simulink model "rfsoc4x2_ospfb_128"  (R2021a)
settings: Solver=VariableStepAuto  StartTime=0.0  StopTime=2048  RelTol=1e-3
undefined symbols (not defined in the file): pfb_coeff_gen_calc
libraries: xbsIndex_r4 x37092, casper_library_delays x737, casper_library_misc x68, xps_library x1
(part 143 of 339)

== system rfsoc4x2_ospfb_128/fft2/fft_direct/butterfly1_0 ==
  a : Inport
  b : Inport  Port=2
  sync_in : Inport  Port=3
  shift : Inport  Port=4
  Concat : xbsIndex_r4/Concat  num_inputs=2  dbl_ovrd=off  block_type=concat
  bus_add : Subsystem  AncestorBlock=casper_library_bus/bus_addsub  mask(bus_addsub){opmode=0, n_bits_a=[18 18], bin_pt_a=17, type_a=1, n_bits_b=[19 19], bin_pt_b=17, type_b=1, cmplx=on, misc=off, async=off, floating_point=off, float_type=single, exp_width=8, frac_width=24, n_bits_out=20, bin_pt_out=17, type_out=1, quantization=0, overflow=0, add_implementation=behavioral HDL, csp_latency=2, pipeline_en=off, pipeline_latency=0}
      mask prompts: opmode "mode (Addition=0, Subtraction=1)"; n_bits_a "a input bit widths"; bin_pt_a "a input binary points"; type_a "a input type (Unsigned=0, Signed=1)"; n_bits_b "b input bit widths"; bin_pt_b "b input binary points"; type_b "b input type (Unsigned=0, Signed=1)"; cmplx "complex"; misc "misc support"; async "asynchronous operation"; floating_point "floating point"; exp_width "exponent width"; frac_width "fraction width"; n_bits_out "output bit widths"; bin_pt_out "output binary points"; type_out "output type (Unsigned=0, Signed=1)"; quantization "quantization strategy (Truncate=0, Round  (unbiased: +/- Inf)=1)"; overflow "overflow strategy (Wrap=0, Saturate=1, Flag as error=2)"; add_implementation "adder implementation"; csp_latency "latency"; pipeline_en "pipeline enable"; pipeline_latency "pipeline latency"
      mask help: Add/subtract components of two busses
      mask init: same as rfsoc4x2_ospfb_128/fft2/fft_direct/butterfly0_0/bus_add
      mask Callback floating_point:
      | onoff = get_param(gcb, 'floating_point');
      | if strcmp(onoff,'on')
      |     enable_fixpt = 'off';
      |     set_param_state(gcb, 'float_type', 'on')
      | 
      |     f_type = get_param(gcb, 'float_type');
      |     if strcmp(f_type,'custom')
      |         set_param_state(gcb, 'exp_width', 'on')
      |         set_param_state(gcb, 'frac_width', 'on')
      |     else
      |         set_param_state(gcb, 'exp_width', 'off')
      |         set_param_state(gcb, 'frac_width', 'off')
      |     end
      | 
      | 
      | else
      |     enable_fixpt = 'on';
      |     set_param_state(gcb, 'float_type', 'off')
      |     set_param_state(gcb, 'exp_width', 'off')
      |     set_param_state(gcb, 'frac_width', 'off')
      | end
      | 
      | set_param_state(gcb, 'n_bits_a', enable_fixpt)
      | set_param_state(gcb, 'bin_pt_a', enable_fixpt)
      | set_param_state(gcb, 'type_a', enable_fixpt)
      | set_param_state(gcb, 'n_bits_b', enable_fixpt)
      | set_param_state(gcb, 'bin_pt_b', enable_fixpt)
      | set_param_state(gcb, 'type_b', enable_fixpt)
      | 
      | set_param_state(gcb, 'n_bits_out', enable_fixpt)
      | set_param_state(gcb, 'bin_pt_out', enable_fixpt)
      | set_param_state(gcb, 'type_out', enable_fixpt)
      | set_param_state(gcb, 'quantization', enable_fixpt)
      | set_param_state(gcb, 'overflow', enable_fixpt)
      mask TypeOptions float_type: single | custom
      mask Callback float_type:
      | f_type = get_param(gcb, 'float_type');
      | if strcmp(f_type,'custom')
      |     set_param_state(gcb, 'exp_width', 'on')
      |     set_param_state(gcb, 'frac_width', 'on')
      | else
      |     set_param_state(gcb, 'exp_width', 'off')
      |     set_param_state(gcb, 'frac_width', 'off')
      | end
      mask TypeOptions add_implementation: behavioral HDL | fabric core | DSP48 core
  bus_convert : Subsystem  AncestorBlock=casper_library_bus/bus_convert  mask(bus_convert){n_bits_in=[21 21 21 21], bin_pt_in=[18 18 18 18], cmplx=on, n_bits_out=18, bin_pt_out=17, quantization=1, overflow=0, csp_latency=conv_latency, of=on, misc=off}
      mask prompts: n_bits_in "input bit widths"; bin_pt_in "input binary points"; cmplx "input complex"; n_bits_out "output bit widths"; bin_pt_out "output binary points"; quantization "quantization strategy (Truncate=0, Round  (unbiased: +/- Inf)=1, Round (unbiased: Even Values)=2)"; overflow "overflow strategy (Wrap=0, Saturate=1, Flag as error=2)"; csp_latency "latency"; of "overflow indication"; misc "misc support"
      mask help: Convert components of busses
      mask init: same as rfsoc4x2_ospfb_128/fft2/fft_direct/butterfly0_0/bus_convert
  bus_expand : Subsystem  AncestorBlock=casper_library_flow_control/bus_expand  mask(bus_expand){mode=divisions of equal size, outputNum=2, outputWidth=[72 72], outputBinaryPt=[0,0], outputArithmeticType=[0,0], show_format=off, outputToWorkspace=off, variablePrefix=out, outputToModelAsWell=on}
      mask prompts: outputNum "Number of outputs:"; outputWidth "Output width:"; outputBinaryPt "Output binary point position:"; outputArithmeticType "Output arithmetic type (ufix=0, fix=1, bool=2):"; show_format "Print format string?"; outputToWorkspace "Output to workspace?"; variablePrefix "Variable name prefix:"; outputToModelAsWell "Output to model as well?"
      mask help:
      | Expands a 'bus' made using a bus_create or Xilinx
      | concat block.
      | The input will be divided into the specified number
      | of outputs with the specified arithmetic types.
      | Divisions are made from most significant bit.
      mask init: same as rfsoc4x2_ospfb_128/bus_expand1
      settings: AttributesFormatString=2 outputs
      mask TypeOptions mode: divisions of equal size | divisions of arbitrary size
      mask Callback mode: %bus_expand_callback();
      mask Callback outputWidth: %bus_expand_callback();
      mask Callback outputToWorkspace: %bus_expand_callback();
  bus_norm0 : Subsystem  AncestorBlock=casper_library_bus/bus_convert  mask(bus_convert){n_bits_in=[20 20 20 20], bin_pt_in=[17 17 17 17], cmplx=on, n_bits_out=21, bin_pt_out=18, quantization=0, overflow=0, csp_latency=0, of=off, misc=off}
      mask prompts: n_bits_in "input bit widths"; bin_pt_in "input binary points"; cmplx "input complex"; n_bits_out "output bit widths"; bin_pt_out "output binary points"; quantization "quantization strategy (Truncate=0, Round  (unbiased: +/- Inf)=1, Round (unbiased: Even Values)=2)"; overflow "overflow strategy (Wrap=0, Saturate=1, Flag as error=2)"; csp_latency "latency"; of "overflow indication"; misc "misc support"
      mask help: Convert components of busses
      mask init: same as rfsoc4x2_ospfb_128/fft2/fft_direct/butterfly0_0/bus_convert
  bus_norm1 : Subsystem  AncestorBlock=casper_library_bus/bus_convert  mask(bus_convert){n_bits_in=[20 20 20 20], bin_pt_in=[18 18 18 18], cmplx=on, n_bits_out=21, bin_pt_out=18, quantization=0, overflow=0, csp_latency=0, of=off, misc=off}
      mask prompts: n_bits_in "input bit widths"; bin_pt_in "input binary points"; cmplx "input complex"; n_bits_out "output bit widths"; bin_pt_out "output binary points"; quantization "quantization strategy (Truncate=0, Round  (unbiased: +/- Inf)=1, Round (unbiased: Even Values)=2)"; overflow "overflow strategy (Wrap=0, Saturate=1, Flag as error=2)"; csp_latency "latency"; of "overflow indication"; misc "misc support"
      mask help: Convert components of busses
      mask init: same as rfsoc4x2_ospfb_128/fft2/fft_direct/butterfly0_0/bus_convert
  bus_relational : Subsystem  AncestorBlock=casper_library_bus/bus_relational  mask(bus_relational){n_bits_a=4, bin_pt_a=0, type_a=0, n_bits_b=[4 4], bin_pt_b=0, type_b=0, en=off, misc=off, mode=a!=b, csp_latency=1}
      mask prompts: n_bits_a "a input bit widths"; bin_pt_a "a input binary points"; type_a "a input type (Unsigned=0, Signed=1)"; n_bits_b "b input bit widths"; bin_pt_b "b input binary points"; type_b "b input type (Unsigned=0, Signed=1)"; en "en port"; misc "misc support"; mode "comparison:"; csp_latency "latency"
      mask help: Find the relational product of two busses
      mask init: same as rfsoc4x2_ospfb_128/fft2/fft_direct/butterfly0_0/bus_relational
      mask TypeOptions mode: a=b | a!=b | a<b | a>b | a<=b | a>=b
  bus_scale : Subsystem  AncestorBlock=casper_library_bus/bus_scale  mask(bus_scale){n_bits_in=[20 20 20 20], bin_pt_in=17, type_in=1, cmplx=on, scale_factor=-1, misc=off}
      mask prompts: n_bits_in "input bit widths"; bin_pt_in "input binary points"; type_in "input types"; cmplx "input complex"; scale_factor "scale factor (2^?)"; misc "misc support"
      mask help: Convert components of busses
      mask init:
      | bus_scale_init(gcb, ...
      |     'n_bits_in', n_bits_in, ...
      |     'bin_pt_in', bin_pt_in, ...
      |     'type_in', type_in, ...
      |     'cmplx', cmplx, ...
      |     'scale_factor', scale_factor, ...
      |     'misc', misc);
  bus_sub : Subsystem  AncestorBlock=casper_library_bus/bus_addsub  mask(bus_addsub){opmode=1, n_bits_a=[18 18], bin_pt_a=17, type_a=1, n_bits_b=[19 19], bin_pt_b=17, type_b=1, cmplx=on, misc=off, async=off, floating_point=off, float_type=single, exp_width=8, frac_width=24, n_bits_out=20, bin_pt_out=17, type_out=1, quantization=0, overflow=0, add_implementation=behavioral HDL, csp_latency=2, pipeline_en=off, pipeline_latency=0}
      mask prompts: opmode "mode (Addition=0, Subtraction=1)"; n_bits_a "a input bit widths"; bin_pt_a "a input binary points"; type_a "a input type (Unsigned=0, Signed=1)"; n_bits_b "b input bit widths"; bin_pt_b "b input binary points"; type_b "b input type (Unsigned=0, Signed=1)"; cmplx "complex"; misc "misc support"; async "asynchronous operation"; floating_point "floating point"; exp_width "exponent width"; frac_width "fraction width"; n_bits_out "output bit widths"; bin_pt_out "output binary points"; type_out "output type (Unsigned=0, Signed=1)"; quantization "quantization strategy (Truncate=0, Round  (unbiased: +/- Inf)=1)"; overflow "overflow strategy (Wrap=0, Saturate=1, Flag as error=2)"; add_implementation "adder implementation"; csp_latency "latency"; pipeline_en "pipeline enable"; pipeline_latency "pipeline latency"
      mask help: Add/subtract components of two busses
      mask init: same as rfsoc4x2_ospfb_128/fft2/fft_direct/butterfly0_0/bus_add
      mask Callback floating_point:
      | onoff = get_param(gcb, 'floating_point');
      | if strcmp(onoff,'on')
      |     enable_fixpt = 'off';
      |     set_param_state(gcb, 'float_type', 'on')
      | 
      |     f_type = get_param(gcb, 'float_type');
      |     if strcmp(f_type,'custom')
      |         set_param_state(gcb, 'exp_width', 'on')
      |         set_param_state(gcb, 'frac_width', 'on')
      |     else
      |         set_param_state(gcb, 'exp_width', 'off')
      |         set_param_state(gcb, 'frac_width', 'off')
      |     end
      | 
      | 
      | else
      |     enable_fixpt = 'on';
      |     set_param_state(gcb, 'float_type', 'off')
      |     set_param_state(gcb, 'exp_width', 'off')
      |     set_param_state(gcb, 'frac_width', 'off')
      | end
      | 
      | set_param_state(gcb, 'n_bits_a', enable_fixpt)
      | set_param_state(gcb, 'bin_pt_a', enable_fixpt)
      | set_param_state(gcb, 'type_a', enable_fixpt)
      | set_param_state(gcb, 'n_bits_b', enable_fixpt)
      | set_param_state(gcb, 'bin_pt_b', enable_fixpt)
      | set_param_state(gcb, 'type_b', enable_fixpt)
      | 
      | set_param_state(gcb, 'n_bits_out', enable_fixpt)
      | set_param_state(gcb, 'bin_pt_out', enable_fixpt)
      | set_param_state(gcb, 'type_out', enable_fixpt)
      | set_param_state(gcb, 'quantization', enable_fixpt)
      | set_param_state(gcb, 'overflow', enable_fixpt)
      mask TypeOptions float_type: single | custom
      mask Callback float_type:
      | f_type = get_param(gcb, 'float_type');
      | if strcmp(f_type,'custom')
      |     set_param_state(gcb, 'exp_width', 'on')
      |     set_param_state(gcb, 'frac_width', 'on')
      | else
      |     set_param_state(gcb, 'exp_width', 'off')
      |     set_param_state(gcb, 'frac_width', 'off')
      | end
      mask TypeOptions add_implementation: behavioral HDL | fabric core | DSP48 core
  constant : xbsIndex_r4/Constant  const=0  gui_display_data_type=Fixed-point  arith_type=Unsigned  n_bits=4  bin_pt=0  preci_type=Single  exp_width=8  frac_width=24  explicit_period=on  period=1  equ=P=C  opselect=C  inp2=PCIN>>17  opr=+  inp1=P  carry=CIN  dbl_ovrd=off  block_type=constant
  delay0 : xbsIndex_r4/Delay  rst=off  infoeditControl=Selection of Reset will increase slice count due to use of real FFs and instead of SRLs  en=off  latency=add_latency+1+conv_latency  reg_retiming=on  dbl_ovrd=off  block_type=delay
  munge : Subsystem  AncestorBlock=casper_library_flow_control/munge  mask(munge){divisions=4, div_size=[2 2 2 2], order=[0 2 1 3], arith_type_out=Unsigned, bin_pt_out=0}
      mask prompts: divisions "Number of divisions"; div_size "Division size (bits)"; order "Division packing order"; arith_type_out "Output arithmetic type"; bin_pt_out "Output binary point"
      mask help: Splits an input bus into the specified number of divisions and then recombines them in the order specified (most significant division = 0,least = number divisions-1)
      mask init:
      | munge_init(gcb, ...
      |     'divisions', divisions, ...
      |     'div_size', div_size, ...
      |     'order', order, ...
      |     'arith_type_out', arith_type_out, ...
      |     'bin_pt_out', bin_pt_out);
      settings: AttributesFormatString=|
      | split:[2 2 2 2]
      | join:[0 2 1 3]
      | Unsigned [8,0]
      mask TypeOptions arith_type_out: Unsigned | Signed  (2's comp) | Floating-point
  mux : Subsystem  AncestorBlock=casper_library_bus/bus_mux  mask(bus_mux){n_inputs=2, n_bits=[21 21 21 21 21 21 21 21], cmplx=off, misc=off, mux_latency=1}
      mask prompts: n_inputs "number of inputs"; n_bits "input bit widths"; cmplx "complex data"; misc "misc support"; mux_latency "mux latency"
      mask help: Mux components of bus
      mask init:
      | bus_mux_init(gcb, ...
      |     'n_inputs', n_inputs, ...
      |     'n_bits', n_bits, ...
      |     'cmplx', cmplx, ...
      |     'misc', misc, ...
      |     'mux_latency', mux_latency);
  shift_replicate : Subsystem  AncestorBlock=casper_library_bus/bus_replicate  mask(bus_replicate){replication=8, csp_latency=1, misc=off, implementation=core}
      mask prompts: replication "replication factor"; csp_latency "latency"; misc "misc support"; implementation "delay implementation"
      mask help: Output bus formed by replicating input bus a number of times
      mask init:
      | bus_replicate_init(gcb, ...
      |     'replication', replication, ...
      |     'csp_latency', csp_latency, ...
      |     'implementation', implementation, ...
      |     'misc', misc);
      mask TypeOptions implementation: core | behavioral
  twiddle : Subsystem  AncestorBlock=casper_library_ffts_twiddle/twiddle_general  mask(twiddle_general){n_inputs=2, FFTSize=9, Coeffs=[0 64 32 96 16 80 48 112 8 72 40 104 24 88 56 120 4 68 36 100 20 84 52 116 12 76 44 108 28 92 60 124 2 66 34 98 18 82 50 114 10 74 42 106 26 90 58 122 6 70 38 102 22 86 54 118 14 78 46 110 30 94 62 126], StepPeriod=0, coeff_bit_width=18, input_bit_width=18, bin_pt_in=17, async=off, floating_point=off, float_type=single, exp_width=8, frac_width=24, add_latency=2, mult_latency=2, bram_latency=2, conv_latency=1, add_pipe_latency=0, mult_pipe_latency=0, coeffs_bit_limit=9, coeff_sharing=off, coeff_decimation=off, coeff_generation=on, cal_bits=9, n_bits_rotation=25, max_fanout=4, use_hdl=on, use_embedded=off, quantization=Round  (unbiased: +/- Inf), overflow=Wrap}
      mask prompts: n_inputs "Number inputs"; FFTSize "FFT Size (2^?)"; Coeffs "Coefficients:"; StepPeriod "Coefficient Step Period (2^?)"; coeff_bit_width "Coefficient Bit Width"; input_bit_width "Input Bit Width"; bin_pt_in "Input binary point"; async "Asynchronous operation"; floating_point "floating point"; float_type "float type"; exp_width "exponent width"; frac_width "fraction width"; add_latency "Add Latency"; mult_latency "Mult Latency"; bram_latency "BRAM Latency"; conv_latency "Convert Latency"; add_pipe_latency "Add Pipeline Latency"; mult_pipe_latency "CMult Pipeline Latency"; coeffs_bit_limit "Number bits above which to store stage's coefficients in BRAM (2^? bits)"; coeff_sharing "BRAM sharing in coeff storage"; coeff_decimation "Store a fraction of coeff factors where useful"; coeff_generation "Generate coeffs with multipliers where useful"; cal_bits "Number calibration locations when generating coeffs (2^?)"; n_bits_rotation "Feedback rotation vector resolution"; max_fanout "Maximum fanout"; use_hdl "Use behavioural HDL for multipliers"; use_embedded "Use embedded multipliers"; quantization "Quantization Behavior"; overflow "Overflow Behavior"
      mask help: Used in biplex pipelined FFT.
      mask init: same as rfsoc4x2_ospfb_128/fft2/fft_direct/butterfly0_0/twiddle
      settings: AttributesFormatString=|
      | data=(18,17)
      | coeffs=(18,17)
      | (Round  (unbiased: +/- Inf),Wrap)
      mask Callback floating_point:
      | onoff = get_param(gcb, 'floating_point');
      | if strcmp(onoff,'on')
      |     enable_fixpt = 'off';
      |     set_param_state(gcb, 'float_type', 'on')
      | 
      |     f_type = get_param(gcb, 'float_type');
      |     if strcmp(f_type,'custom')
      |         set_param_state(gcb, 'exp_width', 'on')
      |         set_param_state(gcb, 'frac_width', 'on')
      |     else
      |         set_param_state(gcb, 'exp_width', 'off')
      |         set_param_state(gcb, 'frac_width', 'off')
      |     end
      | 
      | 
      | else
      |     enable_fixpt = 'on';
      |     set_param_state(gcb, 'float_type', 'off')
      |     set_param_state(gcb, 'exp_width', 'off')
      |     set_param_state(gcb, 'frac_width', 'off')
      | end
      | 
      | set_param_state(gcb, 'input_bit_width', enable_fixpt)
      | set_param_state(gcb, 'bin_pt_in', enable_fixpt)
      | set_param_state(gcb, 'coeff_bit_width', enable_fixpt)
      mask TypeOptions float_type: single | custom
      mask Callback float_type:
      | f_type = get_param(gcb, 'float_type');
      | if strcmp(f_type,'custom')
      |     set_param_state(gcb, 'exp_width', 'on')
      |     set_param_state(gcb, 'frac_width', 'on')
      | else
      |     set_param_state(gcb, 'exp_width', 'off')
      |     set_param_state(gcb, 'frac_width', 'off')
      | end
      mask Callback use_hdl: twiddle_general_callback(gcb);
      mask TypeOptions quantization: Truncate | Round  (unbiased: +/- Inf) | Round  (unbiased: Even Values)
      mask TypeOptions overflow: Wrap | Saturate | Error
      mask DialogControl ParameterTabVar0 Prompt: Basic
      mask DialogControl ParameterTabVar01 Prompt: Latency
      mask DialogControl ParameterTabVar012 Prompt: Implementation
  a+bw : Outport
  a-bw : Outport  Port=2
  of : Outport  Port=3
  sync_out : Outport  Port=4
  wires:
  delay0/1 -> sync_out/1
  twiddle/3(sync_out) -> delay0/1
  bus_relational/1(a!=b) -> of/1
  munge/1(dout) -> bus_relational/2(b)
  constant/1 -> bus_relational/1(a)
  bus_convert/2(overflow) -> munge/1(din)
  bus_expand/2(lsb_out1) -> a-bw/1
  bus_expand/1(msb_out2) -> a+bw/1
  bus_convert/1(dout) -> bus_expand/1(bus_in)
  mux/1(out) -> bus_convert/1(din)
  bus_norm1/1(dout) -> mux/3(d1)
  bus_norm0/1(dout) -> mux/2(d0)
  shift_replicate/1(out) -> mux/1(sel)
  bus_scale/1(dout) -> bus_norm1/1(din)
  Concat/1 -> bus_scale/1(din), bus_norm0/1(din)
  shift/1 -> shift_replicate/1(in)
  bus_sub/1(dout) -> Concat/2
  bus_add/1(dout) -> Concat/1
  twiddle/2(bwo) -> bus_sub/2(b), bus_add/2(b)
  twiddle/1(ao) -> bus_sub/1(a), bus_add/1(a)
  sync_in/1 -> twiddle/3(sync_in)
  b/1 -> twiddle/2(bi)
  a/1 -> twiddle/1(ai)

== system rfsoc4x2_ospfb_128/fft2/fft_direct/butterfly1_1 ==
  a : Inport
  b : Inport  Port=2
  sync_in : Inport  Port=3
  shift : Inport  Port=4
  Concat : xbsIndex_r4/Concat  num_inputs=2  dbl_ovrd=off  block_type=concat
  bus_add : Subsystem  AncestorBlock=casper_library_bus/bus_addsub  mask(bus_addsub){opmode=0, n_bits_a=[18 18], bin_pt_a=17, type_a=1, n_bits_b=[19 19], bin_pt_b=17, type_b=1, cmplx=on, misc=off, async=off, floating_point=off, float_type=single, exp_width=8, frac_width=24, n_bits_out=20, bin_pt_out=17, type_out=1, quantization=0, overflow=0, add_implementation=behavioral HDL, csp_latency=2, pipeline_en=off, pipeline_latency=0}
      mask prompts: opmode "mode (Addition=0, Subtraction=1)"; n_bits_a "a input bit widths"; bin_pt_a "a input binary points"; type_a "a input type (Unsigned=0, Signed=1)"; n_bits_b "b input bit widths"; bin_pt_b "b input binary points"; type_b "b input type (Unsigned=0, Signed=1)"; cmplx "complex"; misc "misc support"; async "asynchronous operation"; floating_point "floating point"; exp_width "exponent width"; frac_width "fraction width"; n_bits_out "output bit widths"; bin_pt_out "output binary points"; type_out "output type (Unsigned=0, Signed=1)"; quantization "quantization strategy (Truncate=0, Round  (unbiased: +/- Inf)=1)"; overflow "overflow strategy (Wrap=0, Saturate=1, Flag as error=2)"; add_implementation "adder implementation"; csp_latency "latency"; pipeline_en "pipeline enable"; pipeline_latency "pipeline latency"
      mask help: Add/subtract components of two busses
      mask init: same as rfsoc4x2_ospfb_128/fft2/fft_direct/butterfly0_0/bus_add
      mask Callback floating_point:
      | onoff = get_param(gcb, 'floating_point');
      | if strcmp(onoff,'on')
      |     enable_fixpt = 'off';
      |     set_param_state(gcb, 'float_type', 'on')
      | 
      |     f_type = get_param(gcb, 'float_type');
      |     if strcmp(f_type,'custom')
      |         set_param_state(gcb, 'exp_width', 'on')
      |         set_param_state(gcb, 'frac_width', 'on')
      |     else
      |         set_param_state(gcb, 'exp_width', 'off')
      |         set_param_state(gcb, 'frac_width', 'off')
      |     end
      | 
      | 
      | else
      |     enable_fixpt = 'on';
      |     set_param_state(gcb, 'float_type', 'off')
      |     set_param_state(gcb, 'exp_width', 'off')
      |     set_param_state(gcb, 'frac_width', 'off')
      | end
      | 
      | set_param_state(gcb, 'n_bits_a', enable_fixpt)
      | set_param_state(gcb, 'bin_pt_a', enable_fixpt)
      | set_param_state(gcb, 'type_a', enable_fixpt)
      | set_param_state(gcb, 'n_bits_b', enable_fixpt)
      | set_param_state(gcb, 'bin_pt_b', enable_fixpt)
      | set_param_state(gcb, 'type_b', enable_fixpt)
      | 
      | set_param_state(gcb, 'n_bits_out', enable_fixpt)
      | set_param_state(gcb, 'bin_pt_out', enable_fixpt)
      | set_param_state(gcb, 'type_out', enable_fixpt)
      | set_param_state(gcb, 'quantization', enable_fixpt)
      | set_param_state(gcb, 'overflow', enable_fixpt)
      mask TypeOptions float_type: single | custom
      mask Callback float_type:
      | f_type = get_param(gcb, 'float_type');
      | if strcmp(f_type,'custom')
      |     set_param_state(gcb, 'exp_width', 'on')
      |     set_param_state(gcb, 'frac_width', 'on')
      | else
      |     set_param_state(gcb, 'exp_width', 'off')
      |     set_param_state(gcb, 'frac_width', 'off')
      | end
      mask TypeOptions add_implementation: behavioral HDL | fabric core | DSP48 core
  bus_convert : Subsystem  AncestorBlock=casper_library_bus/bus_convert  mask(bus_convert){n_bits_in=[21 21 21 21], bin_pt_in=[18 18 18 18], cmplx=on, n_bits_out=18, bin_pt_out=17, quantization=1, overflow=0, csp_latency=conv_latency, of=on, misc=off}
      mask prompts: n_bits_in "input bit widths"; bin_pt_in "input binary points"; cmplx "input complex"; n_bits_out "output bit widths"; bin_pt_out "output binary points"; quantization "quantization strategy (Truncate=0, Round  (unbiased: +/- Inf)=1, Round (unbiased: Even Values)=2)"; overflow "overflow strategy (Wrap=0, Saturate=1, Flag as error=2)"; csp_latency "latency"; of "overflow indication"; misc "misc support"
      mask help: Convert components of busses
      mask init: same as rfsoc4x2_ospfb_128/fft2/fft_direct/butterfly0_0/bus_convert
  bus_expand : Subsystem  AncestorBlock=casper_library_flow_control/bus_expand  mask(bus_expand){mode=divisions of equal size, outputNum=2, outputWidth=[72 72], outputBinaryPt=[0,0], outputArithmeticType=[0,0], show_format=off, outputToWorkspace=off, variablePrefix=out, outputToModelAsWell=on}
      mask prompts: outputNum "Number of outputs:"; outputWidth "Output width:"; outputBinaryPt "Output binary point position:"; outputArithmeticType "Output arithmetic type (ufix=0, fix=1, bool=2):"; show_format "Print format string?"; outputToWorkspace "Output to workspace?"; variablePrefix "Variable name prefix:"; outputToModelAsWell "Output to model as well?"
      mask help:
      | Expands a 'bus' made using a bus_create or Xilinx
      | concat block.
      | The input will be divided into the specified number
      | of outputs with the specified arithmetic types.
      | Divisions are made from most significant bit.
      mask init: same as rfsoc4x2_ospfb_128/bus_expand1
      settings: AttributesFormatString=2 outputs
      mask TypeOptions mode: divisions of equal size | divisions of arbitrary size
      mask Callback mode: %bus_expand_callback();
      mask Callback outputWidth: %bus_expand_callback();
      mask Callback outputToWorkspace: %bus_expand_callback();
  bus_norm0 : Subsystem  AncestorBlock=casper_library_bus/bus_convert  mask(bus_convert){n_bits_in=[20 20 20 20], bin_pt_in=[17 17 17 17], cmplx=on, n_bits_out=21, bin_pt_out=18, quantization=0, overflow=0, csp_latency=0, of=off, misc=off}
      mask prompts: n_bits_in "input bit widths"; bin_pt_in "input binary points"; cmplx "input complex"; n_bits_out "output bit widths"; bin_pt_out "output binary points"; quantization "quantization strategy (Truncate=0, Round  (unbiased: +/- Inf)=1, Round (unbiased: Even Values)=2)"; overflow "overflow strategy (Wrap=0, Saturate=1, Flag as error=2)"; csp_latency "latency"; of "overflow indication"; misc "misc support"
      mask help: Convert components of busses
      mask init: same as rfsoc4x2_ospfb_128/fft2/fft_direct/butterfly0_0/bus_convert
  bus_norm1 : Subsystem  AncestorBlock=casper_library_bus/bus_convert  mask(bus_convert){n_bits_in=[20 20 20 20], bin_pt_in=[18 18 18 18], cmplx=on, n_bits_out=21, bin_pt_out=18, quantization=0, overflow=0, csp_latency=0, of=off, misc=off}
      mask prompts: n_bits_in "input bit widths"; bin_pt_in "input binary points"; cmplx "input complex"; n_bits_out "output bit widths"; bin_pt_out "output binary points"; quantization "quantization strategy (Truncate=0, Round  (unbiased: +/- Inf)=1, Round (unbiased: Even Values)=2)"; overflow "overflow strategy (Wrap=0, Saturate=1, Flag as error=2)"; csp_latency "latency"; of "overflow indication"; misc "misc support"
      mask help: Convert components of busses
      mask init: same as rfsoc4x2_ospfb_128/fft2/fft_direct/butterfly0_0/bus_convert
  bus_relational : Subsystem  AncestorBlock=casper_library_bus/bus_relational  mask(bus_relational){n_bits_a=4, bin_pt_a=0, type_a=0, n_bits_b=[4 4], bin_pt_b=0, type_b=0, en=off, misc=off, mode=a!=b, csp_latency=1}
      mask prompts: n_bits_a "a input bit widths"; bin_pt_a "a input binary points"; type_a "a input type (Unsigned=0, Signed=1)"; n_bits_b "b input bit widths"; bin_pt_b "b input binary points"; type_b "b input type (Unsigned=0, Signed=1)"; en "en port"; misc "misc support"; mode "comparison:"; csp_latency "latency"
      mask help: Find the relational product of two busses
      mask init: same as rfsoc4x2_ospfb_128/fft2/fft_direct/butterfly0_0/bus_relational
      mask TypeOptions mode: a=b | a!=b | a<b | a>b | a<=b | a>=b
  bus_scale : Subsystem  AncestorBlock=casper_library_bus/bus_scale  mask(bus_scale){n_bits_in=[20 20 20 20], bin_pt_in=17, type_in=1, cmplx=on, scale_factor=-1, misc=off}
      mask prompts: n_bits_in "input bit widths"; bin_pt_in "input binary points"; type_in "input types"; cmplx "input complex"; scale_factor "scale factor (2^?)"; misc "misc support"
      mask help: Convert components of busses
      mask init:
      | bus_scale_init(gcb, ...
      |     'n_bits_in', n_bits_in, ...
      |     'bin_pt_in', bin_pt_in, ...
      |     'type_in', type_in, ...
      |     'cmplx', cmplx, ...
      |     'scale_factor', scale_factor, ...
      |     'misc', misc);
  bus_sub : Subsystem  AncestorBlock=casper_library_bus/bus_addsub  mask(bus_addsub){opmode=1, n_bits_a=[18 18], bin_pt_a=17, type_a=1, n_bits_b=[19 19], bin_pt_b=17, type_b=1, cmplx=on, misc=off, async=off, floating_point=off, float_type=single, exp_width=8, frac_width=24, n_bits_out=20, bin_pt_out=17, type_out=1, quantization=0, overflow=0, add_implementation=behavioral HDL, csp_latency=2, pipeline_en=off, pipeline_latency=0}
      mask prompts: opmode "mode (Addition=0, Subtraction=1)"; n_bits_a "a input bit widths"; bin_pt_a "a input binary points"; type_a "a input type (Unsigned=0, Signed=1)"; n_bits_b "b input bit widths"; bin_pt_b "b input binary points"; type_b "b input type (Unsigned=0, Signed=1)"; cmplx "complex"; misc "misc support"; async "asynchronous operation"; floating_point "floating point"; exp_width "exponent width"; frac_width "fraction width"; n_bits_out "output bit widths"; bin_pt_out "output binary points"; type_out "output type (Unsigned=0, Signed=1)"; quantization "quantization strategy (Truncate=0, Round  (unbiased: +/- Inf)=1)"; overflow "overflow strategy (Wrap=0, Saturate=1, Flag as error=2)"; add_implementation "adder implementation"; csp_latency "latency"; pipeline_en "pipeline enable"; pipeline_latency "pipeline latency"
      mask help: Add/subtract components of two busses
      mask init: same as rfsoc4x2_ospfb_128/fft2/fft_direct/butterfly0_0/bus_add
      mask Callback floating_point:
      | onoff = get_param(gcb, 'floating_point');
      | if strcmp(onoff,'on')
      |     enable_fixpt = 'off';
      |     set_param_state(gcb, 'float_type', 'on')
      | 
      |     f_type = get_param(gcb, 'float_type');
      |     if strcmp(f_type,'custom')
      |         set_param_state(gcb, 'exp_width', 'on')
      |         set_param_state(gcb, 'frac_width', 'on')
      |     else
      |         set_param_state(gcb, 'exp_width', 'off')
      |         set_param_state(gcb, 'frac_width', 'off')
      |     end
      | 
      | 
      | else
      |     enable_fixpt = 'on';
      |     set_param_state(gcb, 'float_type', 'off')
      |     set_param_state(gcb, 'exp_width', 'off')
      |     set_param_state(gcb, 'frac_width', 'off')
      | end
      | 
      | set_param_state(gcb, 'n_bits_a', enable_fixpt)
      | set_param_state(gcb, 'bin_pt_a', enable_fixpt)
      | set_param_state(gcb, 'type_a', enable_fixpt)
      | set_param_state(gcb, 'n_bits_b', enable_fixpt)
      | set_param_state(gcb, 'bin_pt_b', enable_fixpt)
      | set_param_state(gcb, 'type_b', enable_fixpt)
      | 
      | set_param_state(gcb, 'n_bits_out', enable_fixpt)
      | set_param_state(gcb, 'bin_pt_out', enable_fixpt)
      | set_param_state(gcb, 'type_out', enable_fixpt)
      | set_param_state(gcb, 'quantization', enable_fixpt)
      | set_param_state(gcb, 'overflow', enable_fixpt)
      mask TypeOptions float_type: single | custom
      mask Callback float_type:
      | f_type = get_param(gcb, 'float_type');
      | if strcmp(f_type,'custom')
      |     set_param_state(gcb, 'exp_width', 'on')
      |     set_param_state(gcb, 'frac_width', 'on')
      | else
      |     set_param_state(gcb, 'exp_width', 'off')
      |     set_param_state(gcb, 'frac_width', 'off')
      | end
      mask TypeOptions add_implementation: behavioral HDL | fabric core | DSP48 core
  constant : xbsIndex_r4/Constant  const=0  gui_display_data_type=Fixed-point  arith_type=Unsigned  n_bits=4  bin_pt=0  preci_type=Single  exp_width=8  frac_width=24  explicit_period=on  period=1  equ=P=C  opselect=C  inp2=PCIN>>17  opr=+  inp1=P  carry=CIN  dbl_ovrd=off  block_type=constant
  delay0 : xbsIndex_r4/Delay  rst=off  infoeditControl=Selection of Reset will increase slice count due to use of real FFs and instead of SRLs  en=off  latency=add_latency+1+conv_latency  reg_retiming=on  dbl_ovrd=off  block_type=delay
  munge : Subsystem  AncestorBlock=casper_library_flow_control/munge  mask(munge){divisions=4, div_size=[2 2 2 2], order=[0 2 1 3], arith_type_out=Unsigned, bin_pt_out=0}
      mask prompts: divisions "Number of divisions"; div_size "Division size (bits)"; order "Division packing order"; arith_type_out "Output arithmetic type"; bin_pt_out "Output binary point"
      mask help: Splits an input bus into the specified number of divisions and then recombines them in the order specified (most significant division = 0,least = number divisions-1)
      mask init:
      | munge_init(gcb, ...
      |     'divisions', divisions, ...
      |     'div_size', div_size, ...
      |     'order', order, ...
      |     'arith_type_out', arith_type_out, ...
      |     'bin_pt_out', bin_pt_out);
      settings: AttributesFormatString=|
      | split:[2 2 2 2]
      | join:[0 2 1 3]
      | Unsigned [8,0]
      mask TypeOptions arith_type_out: Unsigned | Signed  (2's comp) | Floating-point
  mux : Subsystem  AncestorBlock=casper_library_bus/bus_mux  mask(bus_mux){n_inputs=2, n_bits=[21 21 21 21 21 21 21 21], cmplx=off, misc=off, mux_latency=1}
      mask prompts: n_inputs "number of inputs"; n_bits "input bit widths"; cmplx "complex data"; misc "misc support"; mux_latency "mux latency"
      mask help: Mux components of bus
      mask init:
      | bus_mux_init(gcb, ...
      |     'n_inputs', n_inputs, ...
      |     'n_bits', n_bits, ...
      |     'cmplx', cmplx, ...
      |     'misc', misc, ...
      |     'mux_latency', mux_latency);
  shift_replicate : Subsystem  AncestorBlock=casper_library_bus/bus_replicate  mask(bus_replicate){replication=8, csp_latency=1, misc=off, implementation=core}
      mask prompts: replication "replication factor"; csp_latency "latency"; misc "misc support"; implementation "delay implementation"
      mask help: Output bus formed by replicating input bus a number of times
      mask init:
      | bus_replicate_init(gcb, ...
      |     'replication', replication, ...
      |     'csp_latency', csp_latency, ...
      |     'implementation', implementation, ...
      |     'misc', misc);
      mask TypeOptions implementation: core | behavioral
  twiddle : Subsystem  AncestorBlock=casper_library_ffts_twiddle/twiddle_general  mask(twiddle_general){n_inputs=2, FFTSize=9, Coeffs=[1 65 33 97 17 81 49 113 9 73 41 105 25 89 57 121 5 69 37 101 21 85 53 117 13 77 45 109 29 93 61 125 3 67 35 99 19 83 51 115 11 75 43 107 27 91 59 123 7 71 39 103 23 87 55 119 15 79 47 111 31 95 63 127], StepPeriod=0, coeff_bit_width=18, input_bit_width=18, bin_pt_in=17, async=off, floating_point=off, float_type=single, exp_width=8, frac_width=24, add_latency=2, mult_latency=2, bram_latency=2, conv_latency=1, add_pipe_latency=0, mult_pipe_latency=0, coeffs_bit_limit=9, coeff_sharing=off, coeff_decimation=off, coeff_generation=on, cal_bits=9, n_bits_rotation=25, max_fanout=4, use_hdl=on, use_embedded=off, quantization=Round  (unbiased: +/- Inf), overflow=Wrap}
      mask prompts: n_inputs "Number inputs"; FFTSize "FFT Size (2^?)"; Coeffs "Coefficients:"; StepPeriod "Coefficient Step Period (2^?)"; coeff_bit_width "Coefficient Bit Width"; input_bit_width "Input Bit Width"; bin_pt_in "Input binary point"; async "Asynchronous operation"; floating_point "floating point"; float_type "float type"; exp_width "exponent width"; frac_width "fraction width"; add_latency "Add Latency"; mult_latency "Mult Latency"; bram_latency "BRAM Latency"; conv_latency "Convert Latency"; add_pipe_latency "Add Pipeline Latency"; mult_pipe_latency "CMult Pipeline Latency"; coeffs_bit_limit "Number bits above which to store stage's coefficients in BRAM (2^? bits)"; coeff_sharing "BRAM sharing in coeff storage"; coeff_decimation "Store a fraction of coeff factors where useful"; coeff_generation "Generate coeffs with multipliers where useful"; cal_bits "Number calibration locations when generating coeffs (2^?)"; n_bits_rotation "Feedback rotation vector resolution"; max_fanout "Maximum fanout"; use_hdl "Use behavioural HDL for multipliers"; use_embedded "Use embedded multipliers"; quantization "Quantization Behavior"; overflow "Overflow Behavior"
      mask help: Used in biplex pipelined FFT.
      mask init: same as rfsoc4x2_ospfb_128/fft2/fft_direct/butterfly0_0/twiddle
      settings: AttributesFormatString=|
      | data=(18,17)
      | coeffs=(18,17)
      | (Round  (unbiased: +/- Inf),Wrap)
      mask Callback floating_point:
      | onoff = get_param(gcb, 'floating_point');
      | if strcmp(onoff,'on')
      |     enable_fixpt = 'off';
      |     set_param_state(gcb, 'float_type', 'on')
      | 
      |     f_type = get_param(gcb, 'float_type');
      |     if strcmp(f_type,'custom')
      |         set_param_state(gcb, 'exp_width', 'on')
      |         set_param_state(gcb, 'frac_width', 'on')
      |     else
      |         set_param_state(gcb, 'exp_width', 'off')
      |         set_param_state(gcb, 'frac_width', 'off')
      |     end
      | 
      | 
      | else
      |     enable_fixpt = 'on';
      |     set_param_state(gcb, 'float_type', 'off')
      |     set_param_state(gcb, 'exp_width', 'off')
      |     set_param_state(gcb, 'frac_width', 'off')
      | end
      | 
      | set_param_state(gcb, 'input_bit_width', enable_fixpt)
      | set_param_state(gcb, 'bin_pt_in', enable_fixpt)
      | set_param_state(gcb, 'coeff_bit_width', enable_fixpt)
      mask TypeOptions float_type: single | custom
      mask Callback float_type:
      | f_type = get_param(gcb, 'float_type');
      | if strcmp(f_type,'custom')
      |     set_param_state(gcb, 'exp_width', 'on')
      |     set_param_state(gcb, 'frac_width', 'on')
      | else
      |     set_param_state(gcb, 'exp_width', 'off')
      |     set_param_state(gcb, 'frac_width', 'off')
      | end
      mask Callback use_hdl: twiddle_general_callback(gcb);
      mask TypeOptions quantization: Truncate | Round  (unbiased: +/- Inf) | Round  (unbiased: Even Values)
      mask TypeOptions overflow: Wrap | Saturate | Error
      mask DialogControl ParameterTabVar0 Prompt: Basic
      mask DialogControl ParameterTabVar01 Prompt: Latency
      mask DialogControl ParameterTabVar012 Prompt: Implementation
  a+bw : Outport
  a-bw : Outport  Port=2
  of : Outport  Port=3
  sync_out : Outport  Port=4
  wires:
  delay0/1 -> sync_out/1
  twiddle/3(sync_out) -> delay0/1
  bus_relational/1(a!=b) -> of/1
  munge/1(dout) -> bus_relational/2(b)
  constant/1 -> bus_relational/1(a)
  bus_convert/2(overflow) -> munge/1(din)
  bus_expand/2(lsb_out1) -> a-bw/1
  bus_expand/1(msb_out2) -> a+bw/1
  bus_convert/1(dout) -> bus_expand/1(bus_in)
  mux/1(out) -> bus_convert/1(din)
  bus_norm1/1(dout) -> mux/3(d1)
  bus_norm0/1(dout) -> mux/2(d0)
  shift_replicate/1(out) -> mux/1(sel)
  bus_scale/1(dout) -> bus_norm1/1(din)
  Concat/1 -> bus_scale/1(din), bus_norm0/1(din)
  shift/1 -> shift_replicate/1(in)
  bus_sub/1(dout) -> Concat/2
  bus_add/1(dout) -> Concat/1
  twiddle/2(bwo) -> bus_sub/2(b), bus_add/2(b)
  twiddle/1(ao) -> bus_sub/1(a), bus_add/1(a)
  sync_in/1 -> twiddle/3(sync_in)
  b/1 -> twiddle/2(bi)
  a/1 -> twiddle/1(ai)
